simulink model "grid_foll_grid"  (R2024b)
settings: Solver=ode5  StartTime=0.0  StopTime=t_sim  FixedStep=T_sim  MaxStep=1e-4  RelTol=1e-5
values from neighbouring files (symbols this model uses):
  C_2 = 0.05*c_b    (= 1.65327156951e-06)    [init_and_run_perturbed_case.m]
  C_3 = 10*c_b    (= 0.000330654313903)    [init_and_run_perturbed_case.m]
  ext = 1    [init_and_run_perturbed_case.m]
  f_b = 50    [init_and_run_perturbed_case.m]    (also in init_emt2.m)
  L_2 = 0.15*l_b    (= 0.0459639475649)    [init_and_run_perturbed_case.m]
  L_3 = 0.15*l_b    (= 0.0459639475649)    [init_and_run_perturbed_case.m]
  L_f2 = 0.05*l_b    (= 0.015321315855)    [init_and_run_perturbed_case.m]
  R_1 = 2*z_b    (= 192.533333333)    [init_and_run_perturbed_case.m]
  R_2 = 0.015*z_b    (= 1.444)    [init_and_run_perturbed_case.m]
  R_3 = 0.015*z_b    (= 1.444)    [init_and_run_perturbed_case.m]
  T_sample = 2e-4    (= 0.0002)    [init_and_run_perturbed_case.m]    (also in init_emt2.m)
  T_sim = 1e-6    (= 1e-06)    [init_and_run_perturbed_case.m]    (also in init_emt2.m)
  v_b = 380    [init_and_run_perturbed_case.m]    (also in init_emt2.m = 400)
libraries: spsControlledCurrentSourceLib x3, spsGroundLib x3, spsThreePhaseSeriesRLCBranchLib x3, spsThreePhaseParallelRLCBranchLib x1, spsThreePhaseVIMeasurementLib x1, spsThreePhaseSourceLib x1, spspowerguiLib x1
settings Model: Creator=carlo  LastModifiedBy=carlo
settings DataIOCC: ReturnWorkspaceOutputs=off

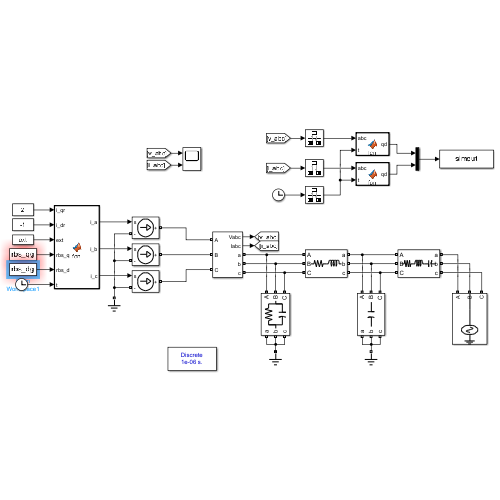
[thumbnail: Simulink's stored preview of the top-level diagram]
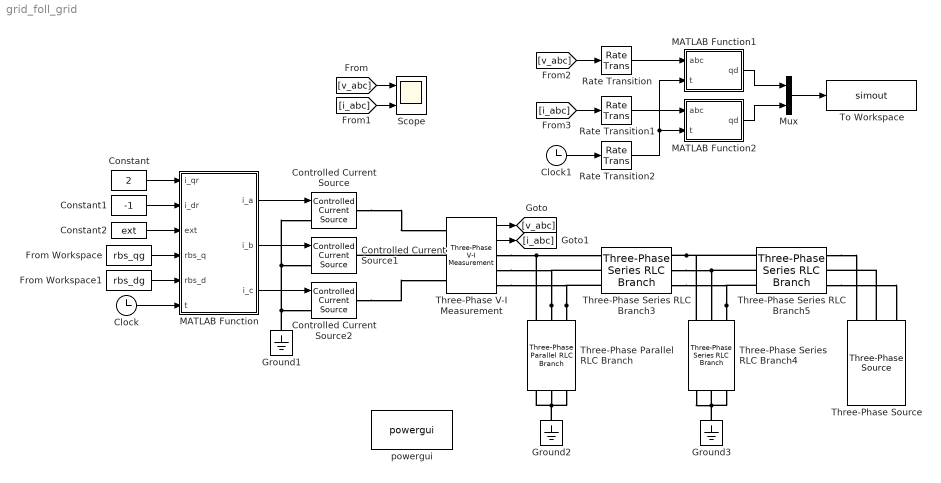
== system grid_foll_grid ==
  Clock : Clock
  Clock1 : Clock
  Constant : Constant  Value=2
  Constant1 : Constant  Value=-1
  Constant2 : Constant  Value=ext
  Controlled Current Source : spsControlledCurrentSourceLib/Controlled Current Source  Initialize=on  Source_Type=AC  Amplitude=0  Phase=0  Frequency=0  Measurements=None
  Controlled Current Source1 : spsControlledCurrentSourceLib/Controlled Current Source  Initialize=on  Source_Type=AC  Amplitude=0  Phase=0  Frequency=0  Measurements=None
  Controlled Current Source2 : spsControlledCurrentSourceLib/Controlled Current Source  Initialize=on  Source_Type=AC  Amplitude=0  Phase=0  Frequency=0  Measurements=None
  From Workspace : FromWorkspace  VariableName=rbs_qg  SampleTime=T_sample
  From Workspace1 : FromWorkspace  VariableName=rbs_dg  SampleTime=T_sample
  Ground1 : spsGroundLib/Ground  LConnTagsString=a
  Ground2 : spsGroundLib/Ground  LConnTagsString=a
  Ground3 : spsGroundLib/Ground  LConnTagsString=a
  MATLAB Function : MATLAB Function  TreatAsAtomicUnit=on
  MATLAB Function1 : MATLAB Function  TreatAsAtomicUnit=on
  MATLAB Function2 : MATLAB Function  TreatAsAtomicUnit=on
  Mux : Mux  Inputs=2
  Rate Transition : RateTransition  OutPortSampleTime=T_sample
  Rate Transition1 : RateTransition  OutPortSampleTime=T_sample
  Rate Transition2 : RateTransition  OutPortSampleTime=T_sample
  Scope : Scope  NumInputPorts=2
  Three-Phase Parallel RLC Branch : spsThreePhaseParallelRLCBranchLib/Three-Phase Parallel RLC Branch  LConnTagsString=A|B|C  RConnTagsString=A|B|C  BranchType=RC  Resistance=R_1  Inductance=1e-3  Capacitance=C_2  Measurements=None
  Three-Phase Series RLC Branch3 : spsThreePhaseSeriesRLCBranchLib/Three-Phase Series RLC Branch  LConnTagsString=A|B|C  RConnTagsString=A|B|C  BranchType=RL  Resistance=R_2  Inductance=L_2  Capacitance=1e-6  Measurements=None
  Three-Phase Series RLC Branch4 : spsThreePhaseSeriesRLCBranchLib/Three-Phase Series RLC Branch  LConnTagsString=A|B|C  RConnTagsString=A|B|C  BranchType=C  Resistance=1  Inductance=L_f2  Capacitance=C_2  Measurements=None
  Three-Phase Series RLC Branch5 : spsThreePhaseSeriesRLCBranchLib/Three-Phase Series RLC Branch  LConnTagsString=A|B|C  RConnTagsString=A|B|C  BranchType=RLC  Resistance=R_3  Inductance=L_3  Capacitance=C_3  Measurements=None
  Three-Phase V-I Measurement : spsThreePhaseVIMeasurementLib/Three-Phase V-I Measurement  VoltageMeasurement=phase-to-ground  SetLabelV=off  LabelV=Vabc  Vpu=off  VpuLL=off  CurrentMeasurement=yes  SetLabelI=off  LabelI=Iabc  Ipu=off  Pbase=100e6  Vbase=500e3  OutputType=Complex  PhasorSimulation=off  PSBequivalent=0
  Three-Phase Source : spsThreePhaseSourceLib/Three-Phase Source  InternalConnection=Yg  VoltagePhases=off  Voltage=v_b  PhaseAngle=90  Voltage_phases=[25e3 25e3 25e3]/sqrt(3)  PhaseAngles_phases=[0 -120 +120]  Frequency=f_b  NonIdealSource=on  SpecifyImpedance=off  Resistance=0.0  Inductance=0.0  ShortCircuitLevel=100e6  BaseVoltage=v_b  XRratio=7  BusType=swing  Pref=10e3  Qref=0  Prefabc=[10e3, 10e3, 10e3]  Qrefabc=[0, 0, 0]  Qmin=-inf  Qmax=inf
  To Workspace : ToWorkspace  VariableName=simout  SaveFormat=Timeseries  SampleTime=-1
  powergui : spspowerguiLib/powergui  Priority=1  SimulationMode=Discrete  SampleTime=T_sim  frequency=60  Iterations=50  frequencyindice=50  Pbase=100e6  ErrMax=1e-4  UnitsV=kV  UnitsW=MW  buscounter=0  FunctionMessages=off  echomessages=off  EnableUseOfTLC=off  CurrentSourceSwitches=off  DisableSnubberDevices=off  DisableRonSwitches=off  DisableVfSwitches=off  DisplayEquations=off  AutomaticDiscreteSolvers=off  SolverType=Tustin/Backward Euler (TBE)  Interpol=off  ExternalGateDelay=off  methode=off  Ts=100  x0status=blocks  SPID=on  SwTol=0  HookPort=off  NonlinearTolerance=1e-4  nMaxIteration=100  ContinueOnMaxIteration=off  RestoreLinks=warning  ResistiveCurrentMeasurement=off  Frange=[0:2:500]  Ylog=off  Xlog=on  ShowGrid=off  save=off  variable=ZData  structure=0  ZoomFFT=off  StartTime=0.0  cycles=1  DisplayStyle=1  fundamental=60  FreqAxis=off  MaxFrequency=1000  frequencyindicesteady=1  RmsSteady=1  display=off
  wires:
  MATLAB Function/1(i_a) -> Controlled Current Source/1
  MATLAB Function/2(i_b) -> Controlled Current Source1/1
  MATLAB Function/3(i_c) -> Controlled Current Source2/1
  From Workspace1/1 -> MATLAB Function/5(rbs_d)
  From Workspace/1 -> MATLAB Function/4(rbs_q)
  Constant/1 -> MATLAB Function/1(i_qr)
  Constant1/1 -> MATLAB Function/2(i_dr)
  Constant2/1 -> MATLAB Function/3(ext)
  Clock/1 -> MATLAB Function/6(t)
  Three-Phase V-I Measurement/1 -> [v_abc]
  Three-Phase V-I Measurement/2 -> [i_abc]
  [v_abc] -> Scope/1
  [i_abc] -> Scope/2
  [v_abc] -> Rate Transition/1
  [i_abc] -> Rate Transition1/1
  Clock1/1 -> Rate Transition2/1
  Rate Transition/1 -> MATLAB Function1/1(abc)
  Rate Transition1/1 -> MATLAB Function2/1(abc)
  Rate Transition2/1 -> MATLAB Function2/2(t), MATLAB Function1/2(t)
  Mux/1 -> To Workspace/1
  MATLAB Function2/1(qd) -> Mux/2
  MATLAB Function1/1(qd) -> Mux/1
  connections:
  Three-Phase V-I Measurement/LConn2 -- Controlled Current Source1/RConn1
  Controlled Current Source/RConn1 -- Three-Phase V-I Measurement/LConn1
  Controlled Current Source2/RConn1 -- Three-Phase V-I Measurement/LConn3
  Three-Phase Series RLC Branch3/RConn1 -- Three-Phase Series RLC Branch4/LConn1 -- Three-Phase Series RLC Branch5/LConn1
  Three-Phase Parallel RLC Branch/RConn2 -- Ground2/LConn1 -- Three-Phase Parallel RLC Branch/RConn1 -- Three-Phase Parallel RLC Branch/RConn3
  Three-Phase Series RLC Branch4/LConn3 -- Three-Phase Series RLC Branch3/RConn3 -- Three-Phase Series RLC Branch5/LConn3
  Three-Phase Parallel RLC Branch/LConn2 -- Three-Phase V-I Measurement/RConn2 -- Three-Phase Series RLC Branch3/LConn2
  Three-Phase Series RLC Branch5/LConn2 -- Three-Phase Series RLC Branch3/RConn2 -- Three-Phase Series RLC Branch4/LConn2
  Three-Phase Series RLC Branch4/RConn2 -- Three-Phase Series RLC Branch4/RConn1 -- Ground3/LConn1 -- Three-Phase Series RLC Branch4/RConn3
  Three-Phase Parallel RLC Branch/LConn3 -- Three-Phase V-I Measurement/RConn3 -- Three-Phase Series RLC Branch3/LConn3
  Three-Phase Source/RConn2 -- Three-Phase Series RLC Branch5/RConn2
  Three-Phase Series RLC Branch5/RConn1 -- Three-Phase Source/RConn1
  Three-Phase Series RLC Branch5/RConn3 -- Three-Phase Source/RConn3
  Three-Phase V-I Measurement/RConn1 -- Three-Phase Parallel RLC Branch/LConn1 -- Three-Phase Series RLC Branch3/LConn1
  Ground1/LConn1 -- Controlled Current Source/LConn1 -- Controlled Current Source1/LConn1 -- Controlled Current Source2/LConn1

== matlab function grid_foll_grid/MATLAB Function1 ==
  data: abc input; qd output; t input
function qd = fcn(abc,t)

w = 100*pi;
th = w*t;
d = 2*pi/3;

Tb = [cos(th), cos(th - d), cos(th + d);
     -sin(th),-sin(th - d),-sin(th + d)];

qd = Tb*abc;

== matlab function grid_foll_grid/MATLAB Function ==
  data: i_qr input; i_a output; i_dr input; ext input; rbs_q input; rbs_d input; t input; i_b output; i_c output
function [i_a, i_b, i_c] = fcn(i_qr, i_dr, ext, rbs_q, rbs_d, t)


i_q = i_qr + ext*rbs_q;
i_d = i_dr + ext*rbs_d;
w = 100*pi;
th = w*t;
d = 2*pi/3;

Tb = [cos(th),     -sin(th);
      cos(th - d), -sin(th -d);
      cos(th + d), -sin(th+d)];

i_abc = Tb*[i_q; i_d];
i_a = i_abc(1);
i_b = i_abc(2);
i_c = i_abc(3);

== matlab function grid_foll_grid/MATLAB Function2 ==
  data: abc input; qd output; t input
function qd = fcn(abc,t)

w = 100*pi;
th = w*t;
d = 2*pi/3;

Tb = [cos(th), cos(th - d), cos(th + d);
     -sin(th),-sin(th - d),-sin(th + d)];

qd = Tb*abc;
